simulink model "TcpReadSend"  (R2026a)
settings: Solver=ode4  StopTime=inf  FixedStep=st
undefined symbols (not defined in the file): Payload
libraries: uavmavlinklib x4, simulink x1
settings Model: Creator=Carlos Fabian  LastModifiedBy=Carlos Fabian
settings ExplorerConfigSet: InternalSimMechanicsExplorerSettings=|
  | <ExplorerConfiguration>
  | 
  |   <canonicalview>default</canonicalview>
  | 
  |   <TilePanel>
  |     <TileInfo>
  |       <Tiles Columns="1" Count="1" Height="513" Rows="1" Width="774">
  |         <Row Weight="1"/>
  |         <Column Weight="1"/>
  |         <Tile Height="1" Width="1" X="0" Y="0"/>
  |       </Tiles>
  |     </TileInfo>
  |     <SceneInfo>
  |       <SceneViewer>
  |         <IsThisViewStd>
  |           <IsStandardView>off</IsStandardView>
  |           <StandardViewName>Front</StandardViewName>
  |         </IsThisViewStd>
  |         <BGColor>
  |           <R>1</R>
  |           <G>1</G>
  |           <B>1</B>
  |           <A>1</A>
  |         </BGColor>
  |         <Camera>
  |           <DoPerspective>off</DoPerspective>
  |           <Position>
  |             <X>16.201091586104312</X>
  |             <Y>-16.65504514146788</Y>
  |             <Z>17.087073385082522</Z>
  |           </Position>
  |           <Center>
  |             <X>-0.25720946651222221</X>
  |             <Y>-0.19674408885134653</Y>
  |             <Z>0.62877233246599318</Z>
  |           </Center>
  |           <Up>
  |             <X>-0.40824829046386302</X>
  |             <Y>0.40824829046386302</Y>
  |             <Z>0.81649658092772615</Z>
  |           </Up>
  |           <XLim>2.5491252053936631</XLim>
  |           <YLim>2.5491252053936631</YLim>
  |           <ViewLimDist>0.01</ViewLimDist>
  |         </Camera>
  |       </SceneViewer>
  |     </SceneInfo>
  |   </TilePanel>
  | 
  |   <MechEditorPanel>
  |     <GfxPanelCameraMap/>
  |     <Cameras/>
  |     <VideoCreator>
  |       <IncludeTiles>All</IncludeTiles>
  |       <IncludeTime>on</IncludeTime>
  |       <IncludeWorldFrame>off</IncludeWorldFrame>
  |       <PlaybackSpeedRatio>8</PlaybackSpeedRatio>
  |       <FrameRate>24</FrameRate>
  |       <FrameSize>auto</FrameSize>
  |       <VideoFormat>MotionJPEGAVI</VideoFormat>
  |     </VideoCreator>
  |   </MechEditorPanel>
  | 
  |   <PlaybackSettings>
  |     <PlaybackSpeedFactor>16</PlaybackSpeedFactor>
  |   </PlaybackSettings>
  | 
  | </ExplorerConfiguration>

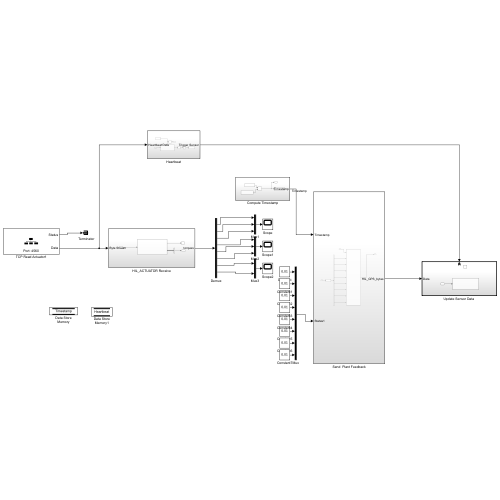
[thumbnail: Simulink's stored preview of the top-level diagram]
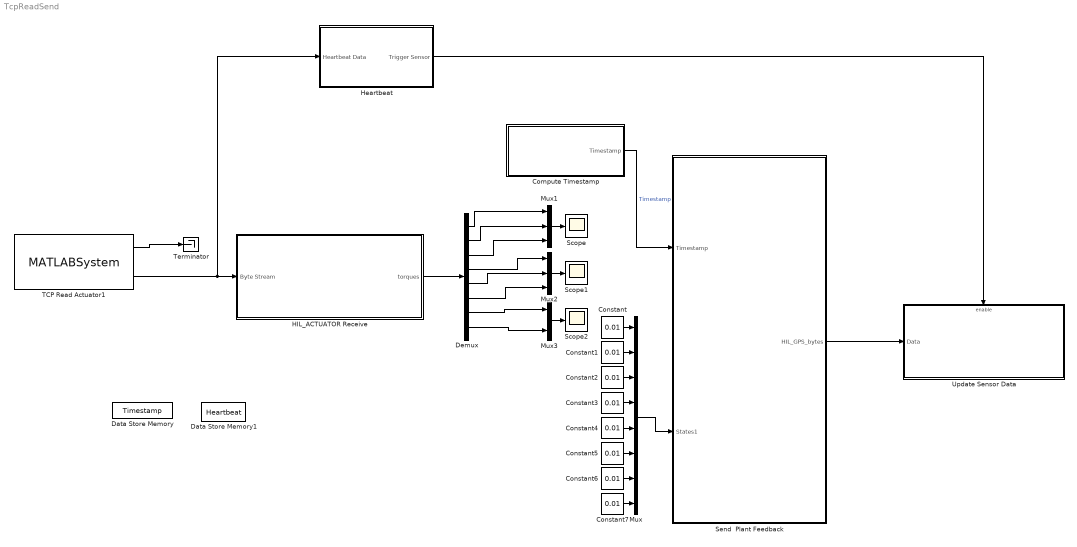
== system TcpReadSend ==
  Compute Timestamp : Subsystem
  Constant{,1..7} (8 alike) : Constant  Value=0.01  SampleTime=0.01
  Data Store Memory : DataStoreMemory  DataStoreName=Timestamp  WriteAfterWriteMsg=warning  ShowAdditionalParam=off
  Data Store Memory1 : DataStoreMemory  DataStoreName=Heartbeat  WriteAfterWriteMsg=warning  InitialValue=1  ShowAdditionalParam=off
  Demux : Demux  Outputs=8
  HIL_ACTUATOR Receive : Subsystem
  Heartbeat : Subsystem
  Mux : Mux  Inputs=8
  Mux1 : Mux  Inputs=3
  Mux2 : Mux  Inputs=3
  Mux3 : Mux  Inputs=2
  Scope : Scope
  Scope1 : Scope
  Scope2 : Scope
      settings: DataLoggingVariableName=ScopeData2
  Send  Plant Feedback : Subsystem
  TCP Read Actuator1 : MATLABSystem  System=px4HostTarget_TCPIP_Read  Length=93  SampleTime=0.01
      mask Type: px4HostTarget_TCPIP_Read
  Terminator : Terminator
  "Update Sensor Data " : Subsystem
  wires:
  TCP Read Actuator1/2 -> Heartbeat/1(Heartbeat Data), HIL_ACTUATOR Receive/1(Byte Stream)
  TCP Read Actuator1/1 -> Terminator/1
  Send  Plant Feedback/1(HIL_GPS_bytes) -> "Update Sensor Data "/1(Data)
  Heartbeat/1(Trigger Sensor) -> "Update Sensor Data "/Enable
  Compute Timestamp/1(Timestamp) -> Send  Plant Feedback/1(Timestamp)  "Timestamp"
  Mux/1 -> Send  Plant Feedback/2(States1)
  Constant/1 -> Mux/1
  Constant1/1 -> Mux/2
  Constant2/1 -> Mux/3
  Constant3/1 -> Mux/4
  Constant4/1 -> Mux/5
  Constant5/1 -> Mux/6
  Constant6/1 -> Mux/7
  Constant7/1 -> Mux/8
  HIL_ACTUATOR Receive/1(torques) -> Demux/1
  Demux/7 -> Mux3/1
  Demux/8 -> Mux3/2
  Demux/6 -> Mux2/3
  Demux/5 -> Mux2/2
  Demux/4 -> Mux2/1
  Demux/3 -> Mux1/3
  Demux/2 -> Mux1/2
  Demux/1 -> Mux1/1
  Mux1/1 -> Scope/1
  Mux2/1 -> Scope1/1
  Mux3/1 -> Scope2/1

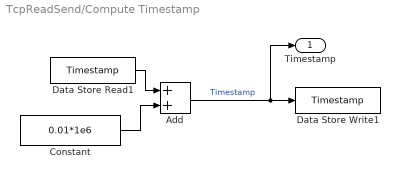
== system TcpReadSend/Compute Timestamp ==
  Add : Sum
  Constant : Constant  Value=0.01*1e6  OutDataTypeStr=uint64  SampleTime=0.01
  Data Store Read1 : DataStoreRead  DataStoreName=Timestamp  SampleTime=0.01  IndexOptions=Index vector (dialog)  Indices=1  OutputSizes=1
  Data Store Write1 : DataStoreWrite  DataStoreName=Timestamp  SampleTime=0.01  IndexOptions=Index vector (dialog)  Indices=1  OutputSizes=1
  Timestamp : Outport
  wires:
  Data Store Read1/1 -> Add/1
  Add/1 -> Data Store Write1/1, Timestamp/1  "Timestamp"
  Constant/1 -> Add/2

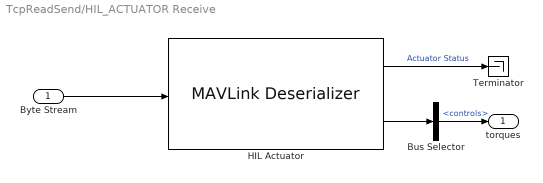
== system TcpReadSend/HIL_ACTUATOR Receive ==
  Byte Stream : Inport
  Bus Selector : BusSelector  OutputSignals=Payload.controls
  HIL Actuator : uavmavlinklib/MAVLink Deserializer  dialectSource=Specify your own  dialect=common.xml  dialectCustom=C:\Users\Carlos Fabian\Documents\MATLAB\UAM_Hexa_PID\mavlink_custom\common.xml  version=2  messageType=HIL_ACTUATOR_CONTROLS  inputDataLength=off  SystemIDFilter=off  systemID=1  ComponentIDFilter=off  componentID=1  queueMsg=off  queueMsgSize=50  dropNum=off
  Terminator : Terminator
  torques : Outport
  wires:
  Byte Stream/1 -> HIL Actuator/1
  HIL Actuator/2 -> Bus Selector/1
  HIL Actuator/1 -> Terminator/1  "Actuator Status"
  Bus Selector/1 -> torques/1  "<controls>"

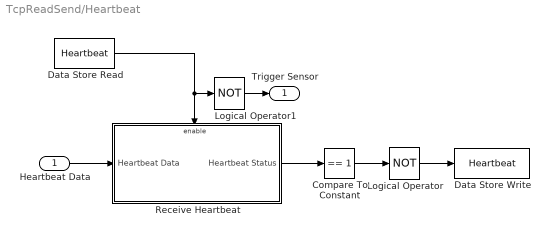
== system TcpReadSend/Heartbeat ==
  Heartbeat Data : Inport
  Compare To Constant : simulink/Logic and Bit Operations/Compare To Constant  relop===  const=1  OutDataTypeStr=uint8
  Data Store Read : DataStoreRead  DataStoreName=Heartbeat  SampleTime=0.01  IndexOptions=Index vector (dialog)  Indices=1  OutputSizes=1
  Data Store Write : DataStoreWrite  DataStoreName=Heartbeat  SampleTime=0.01  IndexOptions=Index vector (dialog)  Indices=1  OutputSizes=1
  Logical Operator : Logic  Operator=NOT  AllPortsSameDT=off  OutDataTypeStr=boolean
  Logical Operator1 : Logic  Operator=NOT  AllPortsSameDT=off  OutDataTypeStr=boolean
  Receive Heartbeat : Subsystem
  Trigger Sensor : Outport
  wires:
  Logical Operator/1 -> Data Store Write/1
  Data Store Read/1 -> Receive Heartbeat/Enable, Logical Operator1/1
  Receive Heartbeat/1(Heartbeat Status) -> Compare To Constant/1
  Compare To Constant/1 -> Logical Operator/1
  Heartbeat Data/1 -> Receive Heartbeat/1(Heartbeat Data)
  Logical Operator1/1 -> Trigger Sensor/1

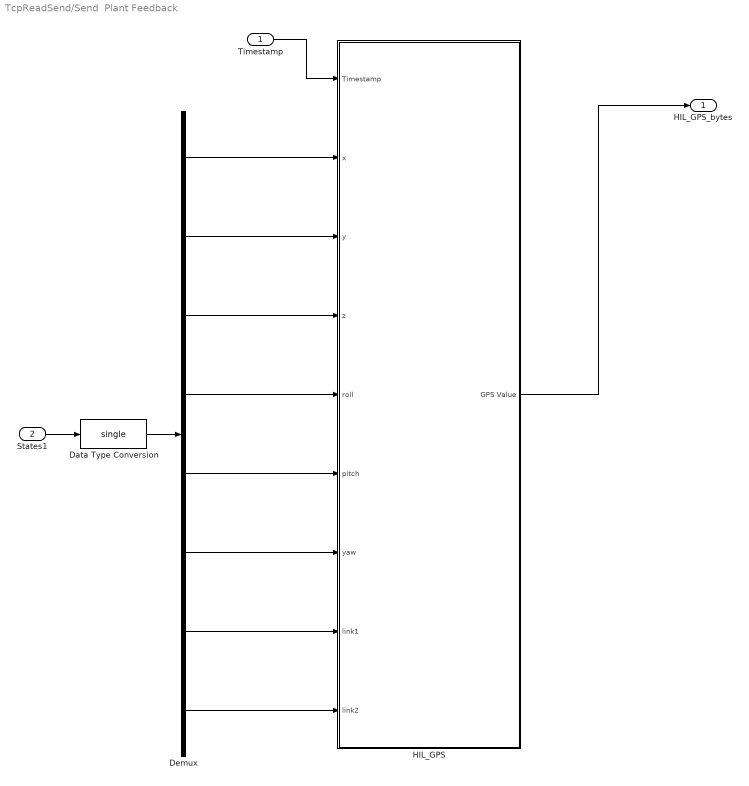
== system TcpReadSend/Send  Plant Feedback ==
  Timestamp : Inport
  States1 : Inport  Port=2
  Data Type Conversion : DataTypeConversion  OutDataTypeStr=single  SaturateOnIntegerOverflow=off  RndMeth=Floor
  Demux : Demux  Outputs=8
  HIL_GPS : Subsystem
  HIL_GPS_bytes : Outport
  wires:
  Timestamp/1 -> HIL_GPS/1(Timestamp)
  HIL_GPS/1(GPS Value) -> HIL_GPS_bytes/1
  States1/1 -> Data Type Conversion/1
  Demux/1 -> HIL_GPS/2(x)
  Demux/2 -> HIL_GPS/3(y)
  Demux/3 -> HIL_GPS/4(z)
  Demux/4 -> HIL_GPS/5(roll)
  Demux/5 -> HIL_GPS/6(pitch)
  Demux/6 -> HIL_GPS/7(yaw)
  Demux/7 -> HIL_GPS/8(link1)
  Demux/8 -> HIL_GPS/9(link2)
  Data Type Conversion/1 -> Demux/1

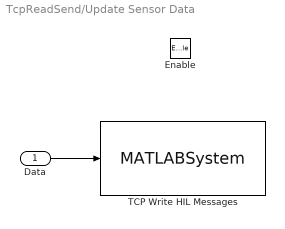
== system TcpReadSend/Update Sensor Data  ==
  Data : Inport
  Enable : EnablePort
  TCP Write HIL Messages : MATLABSystem  System=px4HostTarget_TCPIP_Write
      mask Type: px4HostTarget_TCPIP_Write
  wires:
  Data/1 -> TCP Write HIL Messages/1

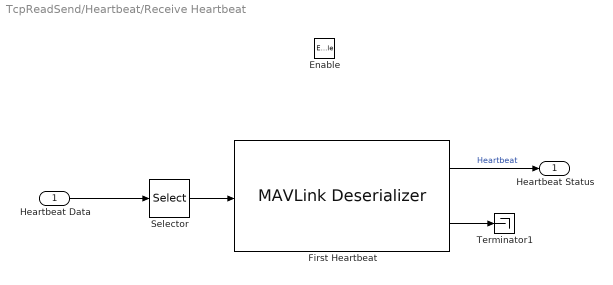
== system TcpReadSend/Heartbeat/Receive Heartbeat ==
  Heartbeat Data : Inport
  Enable : EnablePort
  First Heartbeat : uavmavlinklib/MAVLink Deserializer  dialectSource=Specify your own  dialect=common.xml  dialectCustom=C:\Users\Carlos Fabian\Documents\MATLAB\UAM_Hexa_PID\mavlink_custom\common.xml  version=2  messageType=HEARTBEAT  inputDataLength=off  SystemIDFilter=off  systemID=1  ComponentIDFilter=off  componentID=1  queueMsg=off  queueMsgSize=50  dropNum=off
  Selector : Selector  InputPortWidth=93  IndexOptions=Index vector (dialog)  Indices=[1:63]  OutputSizes=1
  Terminator1 : Terminator
  Heartbeat Status : Outport
  wires:
  First Heartbeat/2 -> Terminator1/1
  Selector/1 -> First Heartbeat/1
  First Heartbeat/1 -> Heartbeat Status/1  "Heartbeat"
  Heartbeat Data/1 -> Selector/1

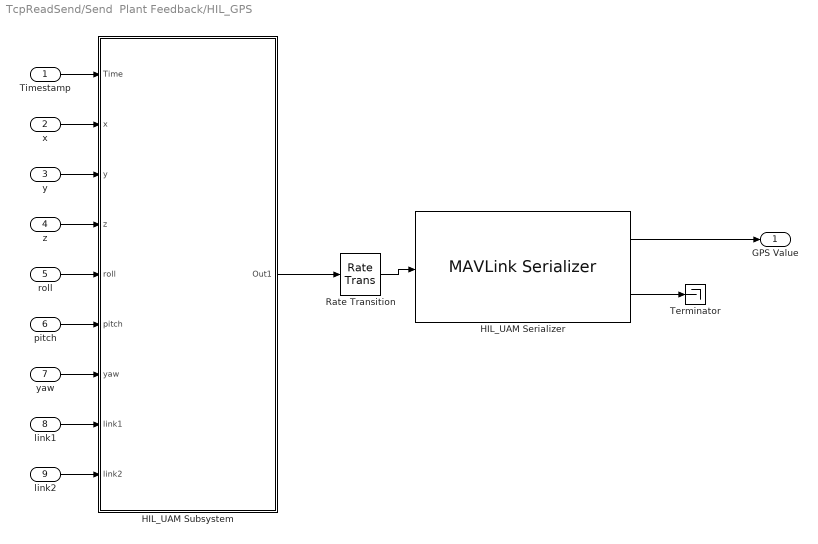
== system TcpReadSend/Send  Plant Feedback/HIL_GPS ==
  Timestamp : Inport
  x : Inport  Port=2
  y : Inport  Port=3
  z : Inport  Port=4
  roll : Inport  Port=5
  pitch : Inport  Port=6
  yaw : Inport  Port=7
  link1 : Inport  Port=8
  link2 : Inport  Port=9
  HIL_UAM Serializer : uavmavlinklib/MAVLink Serializer  dialectSource=Specify your own  dialect=common.xml  dialectCustom=C:\Users\Carlos Fabian\Documents\MATLAB\UAM_Hexa_PID\mavlink_custom\common.xml  version=2  messageType=UAM_STATES
  HIL_UAM Subsystem : Subsystem
  Rate Transition : RateTransition  OutPortSampleTime=0.01
  Terminator : Terminator
  GPS Value : Outport
  wires:
  Timestamp/1 -> HIL_UAM Subsystem/1(Time)
  x/1 -> HIL_UAM Subsystem/2(x)
  y/1 -> HIL_UAM Subsystem/3(y)
  z/1 -> HIL_UAM Subsystem/4(z)
  yaw/1 -> HIL_UAM Subsystem/7(yaw)
  pitch/1 -> HIL_UAM Subsystem/6(pitch)
  roll/1 -> HIL_UAM Subsystem/5(roll)
  link2/1 -> HIL_UAM Subsystem/9(link2)
  link1/1 -> HIL_UAM Subsystem/8(link1)
  HIL_UAM Subsystem/1(Out1) -> Rate Transition/1
  HIL_UAM Serializer/2 -> Terminator/1
  HIL_UAM Serializer/1 -> GPS Value/1
  Rate Transition/1 -> HIL_UAM Serializer/1

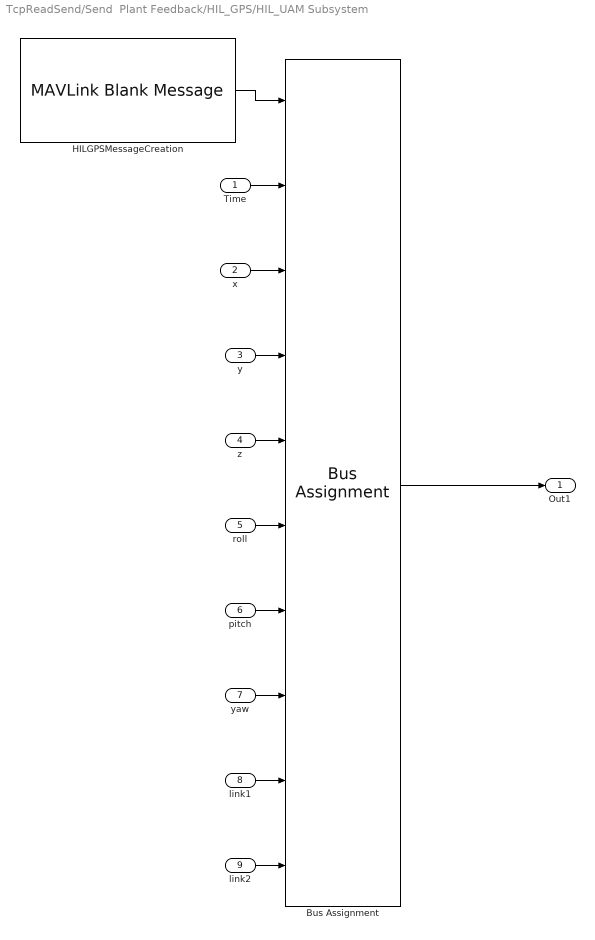
== system TcpReadSend/Send  Plant Feedback/HIL_GPS/HIL_UAM Subsystem ==
  Time : Inport
  x : Inport  Port=2
  y : Inport  Port=3
  z : Inport  Port=4
  roll : Inport  Port=5
  pitch : Inport  Port=6
  yaw : Inport  Port=7
  link1 : Inport  Port=8
  link2 : Inport  Port=9
  Bus Assignment : BusAssignment  AssignedSignals=Payload.time_usec,Payload.pos_x,Payload.pos_y,Payload.pos_z,Payload.roll,Payload.pitch,Payload.yaw,Payload.link_one,Payload.link_two
  HILGPSMessageCreation : uavmavlinklib/MAVLink Blank Message  dialectSource=Specify your own  dialect=common.xml  dialectCustom=C:\Users\Carlos Fabian\Documents\MATLAB\UAM_Hexa_PID\mavlink_custom\common.xml  version=2  messageType=UAM_STATES  SystemID=2  ComponentID=51  SampleTime=0.01
  Out1 : Outport
  wires:
  HILGPSMessageCreation/1 -> Bus Assignment/1
  Bus Assignment/1 -> Out1/1
  Time/1 -> Bus Assignment/2
  roll/1 -> Bus Assignment/6
  yaw/1 -> Bus Assignment/8
  pitch/1 -> Bus Assignment/7
  x/1 -> Bus Assignment/3
  y/1 -> Bus Assignment/4
  z/1 -> Bus Assignment/5
  link1/1 -> Bus Assignment/9
  link2/1 -> Bus Assignment/10
